simulink model "ArduPlane_LindiPlane"  (R2023b)
settings: Solver=FixedStepDiscrete  StartTime=0.0  StopTime=1000  FixedStep=double(lindi_notune.ts)  RelTol=1e-4
libraries: ardupilot_custom_controller_lib x2, simulink x2, lindiPlane_lib x1, axes_transformation_lib x1
settings Model: DataTypeOverride=Single  DataTypeOverrideAppliesTo=Floating-point  TunableVars=lindi  TunableVarsStorageClass=Auto  Creator=Yannic  LastModifiedBy=yannic
settings SolverCC: ZeroCrossControl=DisableAll  AlgebraicLoopSolver=TrustRegion
settings DataIOCC: LimitDataPoints=on  SaveOutput=off  SaveTime=off
settings OptimizationCC: DefaultParameterBehavior=Inlined  UseDivisionForNetSlopeComputation=on  UseFloatMulNetSlope=on  DefaultUnderspecifiedDataType=single  InlineInvariantSignals=on  ReuseModelBlockBuffer=off  PassReuseOutputArgsAs=Individual arguments  ZeroExternalMemoryAtStartup=off  ZeroInternalMemoryAtStartup=off  NoFixptDivByZeroProtection=on  EfficientFloat2IntCast=on  LifeSpan=1  OptimizationLevel=level1  OptimizationCustomize=off  EfficientTunableParamExpr=on
settings DebuggingCC: ReadBeforeWriteMsg=DisableAll  WriteAfterWriteMsg=DisableAll  WriteAfterReadMsg=DisableAll  MultiTaskDSMMsg=none  ParameterTunabilityLossMsg=error  UnconnectedInputMsg=warning  UnconnectedOutputMsg=warning  UnconnectedLineMsg=warning  AllowSymbolicDim=off  SFUnexpectedBacktrackingDiag=warning  SFNoUnconditionalDefaultTransitionDiag=warning  SFExecutionAtInitializationDiag=none  ArithmeticOperatorsInVariantConditions=warning
settings HardwareCC: ProdBitPerLong=64  ProdLongLongMode=on  ProdHWDeviceType=Intel->x86-64 (Linux 64)
settings ModelReferenceCC: UpdateModelReferenceTargets=IfOutOfDate  EnableRefExpFcnMdlSchedulingChecks=on  PropagateSignalLabelsOutOfModel=off
settings SFSimCC: SFSimEcho=off  SimUseLocalCustomCode=off  MATLABDynamicMemAlloc=off  CustomCodeUndefinedFunction=UseInterfaceOnly  SimTargetLang=C++
settings RTWCC: Description=Embedded Coder  SystemTargetFile=ert.tlc  GenCodeOnly=on  TemplateMakefile=ert_default_tmf  GenerateReport=on  RTWUseLocalCustomCode=off  CustomSourceCode=//custom_source_file_import_identifier  CustomHeaderCode=//custom_header_file_import_identifier  IncludeHyperlinkInReport=on  LaunchReport=on  TargetLang=C++  GenerateTraceInfo=on  GenerateTraceReport=on  GenerateTraceReportSl=on  GenerateTraceReportSf=on  GenerateTraceReportEml=on
settings CodeAppCC: ForceParamTrailComments=on  IgnoreCustomStorageClasses=off  OperatorAnnotations=on  SimulinkDataObjDesc=on  SFDataObjDesc=on  CustomSymbolStrGlobalVar=rt$N$M  CustomSymbolStrType=$N$M  CustomSymbolStrFcn=$N$M$F  CustomSymbolStrMacro=$N$M  InsertBlockDesc=on
settings ERTTargetCC: TargetLangStandard=C++03 (ISO)  IncludeMdlTerminateFcn=off  CombineSignalStateStructs=on  SuppressErrorStatus=on  SupportAbsoluteTime=off  CodeInterfacePackaging=C++ class  SupportNonFinite=off  SupportComplex=off  SupportVariableSizeSignals=on  ERTHeaderFileRootName=MatlabController$E  ERTSourceFileRootName=MatlabController$E  ERTDataFileRootName=MatlabController_data  InlinedParameterPlacement=NonHierarchical  RootIOFormat=Structure reference  ERTCustomFileTemplate=example_file_process.tlc  ERTFilePackagingFormat=CompactWithDataFile
settings ConfigComp: CovMetricSettings=dw  CovSaveCumulativeToWorkspaceVar=on  CovSaveSingleToWorkspaceVar=on  CovExternalEMLEnable=off

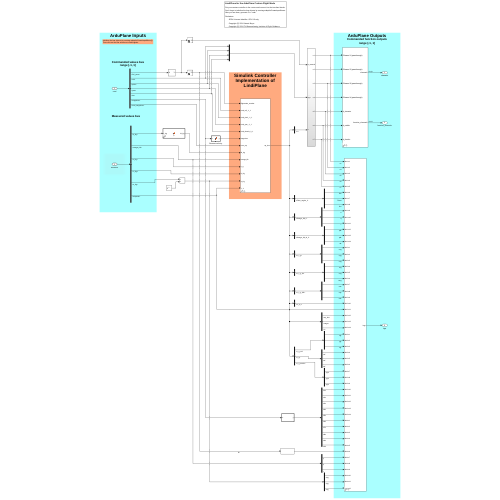
[thumbnail: Simulink's stored preview of the top-level diagram]
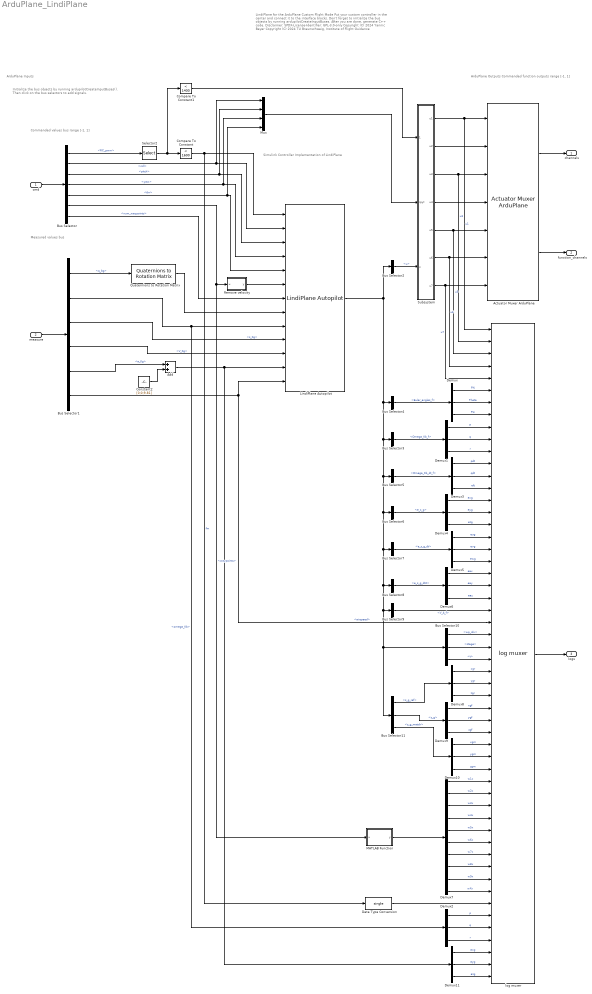
== system ArduPlane_LindiPlane ==
  note: Measured values bus
  note: Initialize the bus objects by running ardupilotCreateInputBuses().
      | Then click on the bus selectors to add signals.
  note: Commanded values bus
      | range [-1, 1]
  note: ArduPlane Inputs
  note: ArduPlane Outputs
      | Commanded function outputs
      | range [-1, 1]
  note: Simulink Controller
      | Implementation of
      | LindiPlane
  note: LindiPlane for the ArduPlane Custom Flight Mode
      |
      | Put your custom controller in the center and connect it to the interface blocks.
      | Don't forget to initialize the bus objects by running ardupilotCreateInputBuses.
      | After you are done, generate C++ code.
      |
      | Disclaimer:
      | SPDX-License-Identifier: GPL-3.0-only
      |
      | Copyright (C) 2024 Yannic Beyer
      | Copyright (C) 2024 TU Braunschweig, Institute of Flight Guidance
  cmd : Inport  OutDataTypeStr=Bus: cmdBus
  measure : Inport  Port=2  OutDataTypeStr=Bus: measureBus
  Actuator Muxer ArduPlane : ardupilot_custom_controller_lib/Actuator Muxer ArduPlane  num_channels=7  CHFCN1=passthrough  CHFCN2=passthrough  CHFCN3=passthrough  CHFCN4=passthrough  CHFCN5=k_elevator  CHFCN6=k_rudder  CHFCN7=k_throttle  CHFCN8=passthrough  CHFCN9=k_elevator  CHFCN10=k_rudder  CHFCN11=k_throttle  CHFCN12=k_none  CHFCN13=k_none  CHFCN14=k_none  CHFCN15=k_none  CHFCN16=k_none
      settings: SourceProductName=LADAC
  Add : Sum
  Bus Selector : BusSelector  OutputSignals=RC_pwm,roll,pitch,yaw,thr,waypoints,num_waypoints
  Bus Selector1 : BusSelector  OutputSignals=q_bg,omega_Kb,s_Kg,V_Kg,a_Kg,airspeed
  Bus Selector10 : BusSelector  OutputSignals=wpnav.wp_idx,wpnav.stage,wpnav.t
  Bus Selector11 : BusSelector  OutputSignals=pos_control.reference.s_g_ref,pos_control.measure.s_g,wpnav.s_g_match
  Bus Selector2 : BusSelector  OutputSignals=inner_loop_indi.u
  Bus Selector3 : BusSelector  OutputSignals=measurements.Omega_Kb_f
  Bus Selector4 : BusSelector  OutputSignals=measurements.Euler_angles_f
  Bus Selector5 : BusSelector  OutputSignals=measurements.Omega_Kb_dt_f
  Bus Selector6 : BusSelector  OutputSignals=pos_control.error.e_s_g
  Bus Selector7 : BusSelector  OutputSignals=pos_control.error.e_s_g_dt
  Bus Selector8 : BusSelector  OutputSignals=pos_control.error.e_s_g_dt2
  Bus Selector9 : BusSelector  OutputSignals=measurements.V_A_f
  Compare To Constant : simulink/Logic and Bit Operations/Compare To Constant  relop=<  const=1600  OutDataTypeStr=uint8
  Compare To Constant1 : simulink/Logic and Bit Operations/Compare To Constant  relop=<  const=1400  OutDataTypeStr=boolean
  Constant2 : Constant  Value=[0;0;9.81]  OutDataTypeStr=Inherit: Inherit via back propagation
  Data Type Conversion : DataTypeConversion  OutDataTypeStr=single  SaturateOnIntegerOverflow=off  RndMeth=Floor
  Demux{,1..6,8..11} (11 alike) : Demux  Outputs=3
  Demux7 : Demux  Outputs=10
  LindiPlane Autopilot : lindiPlane_lib/LindiPlane Autopilot  ap=lindi  ap_notune=lindi_notune  is_enable_checked=off  states_when_enabling=reset  is_cmd_wrbm_n=off
  MATLAB Function : MATLAB Function  TreatAsAtomicUnit=on
  Mux : Mux
  Quaternions to Rotation Matrix : axes_transformation_lib/Quaternions to Rotation Matrix  SystemSampleTime=-1  VariantActivationTime=update diagram  AllowFlexibleInterface=on  Latency=0  AutoFrameSizeCalculation=off
      settings: SourceProductName=LADAC
  Remove velocity : MATLAB Function  TreatAsAtomicUnit=on
  Selector2 : Selector  InputPortWidth=16  IndexOptions=Index vector (dialog)  Indices=8  OutputSizes=1
  Subsystem : Subsystem
  log muxer : ardupilot_custom_controller_lib/log muxer  batch_name_1='ML1'  num_signals_1=14  batch_name_2='ML2'  num_signals_2=14  batch_name_3='ML3'  num_signals_3=14  batch_name_4='ML4'  num_signals_4=12  batch_name_5='ML5'  num_signals_5=0
      settings: SourceProductName=LADAC
  channels : Outport  VectorParamsAs1DForOutWhenUnconnected=off
  function_channels : Outport  Port=2  VectorParamsAs1DForOutWhenUnconnected=off
  logs : Outport  Port=3  VectorParamsAs1DForOutWhenUnconnected=off
  wires:
  cmd/1 -> Bus Selector/1
  measure/1 -> Bus Selector1/1
  Bus Selector1/2 -> LindiPlane Autopilot/9, Demux2/1  "<omega_Kb>"
  Bus Selector/2 -> LindiPlane Autopilot/2, Mux/1  "<roll>"
  Bus Selector/3 -> LindiPlane Autopilot/3, Mux/2  "<pitch>"
  Bus Selector/4 -> LindiPlane Autopilot/4, Mux/3  "<yaw>"
  Bus Selector/5 -> LindiPlane Autopilot/5, Mux/4  "<thr>"
  Bus Selector1/4 -> LindiPlane Autopilot/11  "<V_Kg>"
  log muxer/1 -> logs/1
  Demux/1 -> log muxer/6  "Phi"
  Demux/2 -> log muxer/7  "Theta"
  Demux/3 -> log muxer/8  "Psi"
  Demux1/1 -> log muxer/9  "p"
  Demux1/2 -> log muxer/10  "q"
  Demux1/3 -> log muxer/11  "r"
  Demux3/1 -> log muxer/12  "pdt"
  Demux3/2 -> log muxer/13  "qdt"
  Demux3/3 -> log muxer/14  "rdt"
  Actuator Muxer ArduPlane/1 -> channels/1
  Actuator Muxer ArduPlane/2 -> function_channels/1
  Bus Selector1/1 -> Quaternions to Rotation Matrix/1  "<q_bg>"
  Quaternions to Rotation Matrix/1 -> LindiPlane Autopilot/8
  Bus Selector1/3 -> LindiPlane Autopilot/10  "<s_Kg>"
  Bus Selector1/5 -> Add/1  "<a_Kg>"
  Bus Selector1/6 -> LindiPlane Autopilot/13, log muxer/25  "<airspeed>"
  Bus Selector/6 -> MATLAB Function/1(u), Remove velocity/1(u)  "<waypoints>"
  LindiPlane Autopilot/1 -> Bus Selector11/1, Bus Selector10/1, Bus Selector9/1, Bus Selector8/1, Bus Selector7/1, Bus Selector6/1, Bus Selector5/1, Bus Selector3/1, Bus Selector4/1, Bus Selector2/1
  Bus Selector4/1 -> Demux/1  "<Euler_angles_f>"
  Bus Selector3/1 -> Demux1/1  "<Omega_Kb_f>"
  Bus Selector5/1 -> Demux3/1  "<Omega_Kb_dt_f>"
  Demux4/1 -> log muxer/15  "exg"
  Demux4/2 -> log muxer/16  "eyg"
  Demux4/3 -> log muxer/17  "ezg"
  Bus Selector6/1 -> Demux4/1  "<e_s_g>"
  Demux5/1 -> log muxer/18  "eug"
  Demux5/2 -> log muxer/19  "evg"
  Demux5/3 -> log muxer/20  "ewg"
  Bus Selector7/1 -> Demux5/1  "<e_s_g_dt>"
  Demux6/1 -> log muxer/21  "eax"
  Demux6/2 -> log muxer/22  "eay"
  Demux6/3 -> log muxer/23  "eaz"
  Bus Selector8/1 -> Demux6/1  "<e_s_g_dt2>"
  Bus Selector9/1 -> log muxer/24  "<V_A_f>"
  Bus Selector/1 -> Selector2/1  "<RC_pwm>"
  Compare To Constant/1 -> LindiPlane Autopilot/1, Data Type Conversion/1  "fm"
  Remove velocity/1(y) -> LindiPlane Autopilot/6
  Selector2/1 -> Compare To Constant1/1, Compare To Constant/1
  Bus Selector2/1 -> Subsystem/3(u)  "<u>"
  Subsystem/7(u7) -> log muxer/5, Actuator Muxer ArduPlane/7  "u7"
  Subsystem/4(u4) -> Actuator Muxer ArduPlane/4
  Subsystem/3(u3) -> log muxer/2, Actuator Muxer ArduPlane/3  "u3"
  Subsystem/2(u2) -> Actuator Muxer ArduPlane/2
  Subsystem/1(u1) -> Actuator Muxer ArduPlane/1, log muxer/1  "u1"
  Subsystem/5(u5) -> log muxer/3, Actuator Muxer ArduPlane/5  "u5"
  Subsystem/6(u6) -> log muxer/4, Actuator Muxer ArduPlane/6  "u6"
  Mux/1 -> Subsystem/2(rpyt)
  Compare To Constant1/1 -> Subsystem/1(is_manual)
  MATLAB Function/1(y) -> Demux7/1
  Constant2/1 -> Add/2
  Add/1 -> Demux11/1, LindiPlane Autopilot/12
  Demux2/3 -> log muxer/51  "r"
  Demux2/2 -> log muxer/50  "q"
  Demux2/1 -> log muxer/49  "p"
  Demux7/10 -> log muxer/47  "wXx"
  Demux7/9 -> log muxer/46  "w9x"
  Demux7/8 -> log muxer/45  "w8x"
  Demux7/7 -> log muxer/44  "w7x"
  Demux7/6 -> log muxer/43  "w6x"
  Demux7/5 -> log muxer/42  "w5x"
  Demux7/4 -> log muxer/41  "w4x"
  Demux7/3 -> log muxer/40  "w3x"
  Demux7/2 -> log muxer/39  "w2x"
  Demux7/1 -> log muxer/38  "w1x"
  Data Type Conversion/1 -> log muxer/48
  Bus Selector10/1 -> log muxer/26  "<wp_idx>"
  Bus Selector10/2 -> log muxer/27  "<stage>"
  Bus Selector10/3 -> log muxer/28  "<t>"
  Bus Selector11/1 -> Demux8/1  "<s_g_ref>"
  Demux8/1 -> log muxer/29  "xgr"
  Demux8/2 -> log muxer/30  "ygr"
  Demux8/3 -> log muxer/31  "zgr"
  Demux9/1 -> log muxer/32  "xgf"
  Demux9/2 -> log muxer/33  "ygf"
  Demux9/3 -> log muxer/34  "zgf"
  Bus Selector11/2 -> Demux9/1  "<s_g>"
  Demux10/1 -> log muxer/35  "xgm"
  Demux10/2 -> log muxer/36  "ygm"
  Demux10/3 -> log muxer/37  "zgm"
  Bus Selector11/3 -> Demux10/1  "<s_g_match>"
  Bus Selector/7 -> LindiPlane Autopilot/7  "<num_waypoints>"
  Demux11/3 -> log muxer/54  "azg"
  Demux11/2 -> log muxer/53  "ayg"
  Demux11/1 -> log muxer/52  "axg"

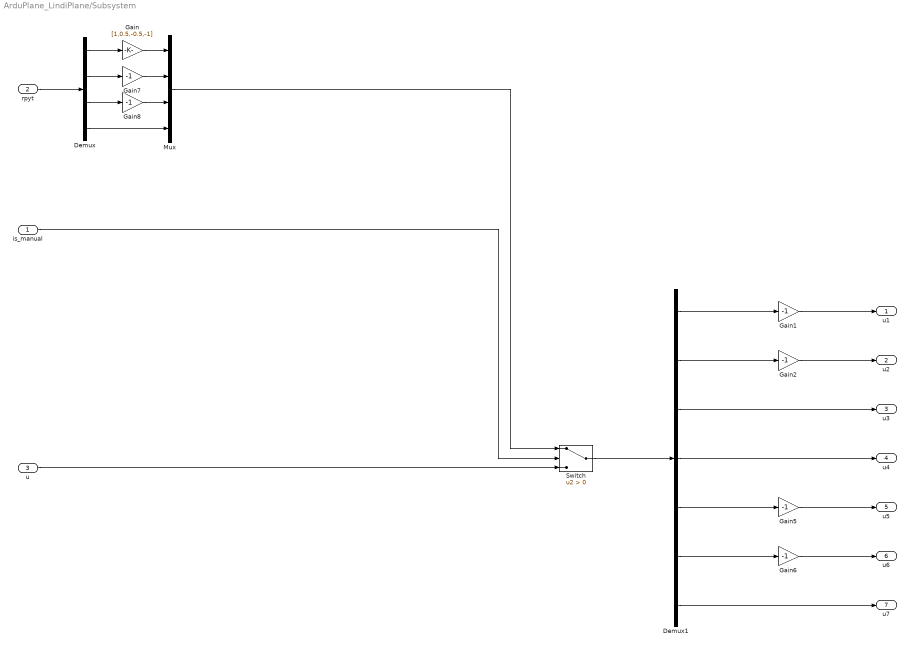
== system ArduPlane_LindiPlane/Subsystem ==
  is_manual : Inport
  rpyt : Inport  Port=2
  u : Inport  Port=3
  Demux : Demux
  Demux1 : Demux  Outputs=7
  Gain : Gain  Gain=[1,0.5,-0.5,-1]
  Gain{1..2,5..8} (6 alike) : Gain  Gain=-1
  Mux : Mux
  Switch : Switch  Criteria=u2 > Threshold  SaturateOnIntegerOverflow=off  InputSameDT=off
  u1 : Outport  VectorParamsAs1DForOutWhenUnconnected=off
  u2 : Outport  Port=2  VectorParamsAs1DForOutWhenUnconnected=off
  u3 : Outport  Port=3  VectorParamsAs1DForOutWhenUnconnected=off
  u4 : Outport  Port=4  VectorParamsAs1DForOutWhenUnconnected=off
  u5 : Outport  Port=5  VectorParamsAs1DForOutWhenUnconnected=off
  u6 : Outport  Port=6  VectorParamsAs1DForOutWhenUnconnected=off
  u7 : Outport  Port=7  VectorParamsAs1DForOutWhenUnconnected=off
  wires:
  is_manual/1 -> Switch/2
  rpyt/1 -> Demux/1
  Demux/1 -> Gain/1
  Demux/4 -> Mux/4
  Demux/3 -> Gain8/1
  Demux/2 -> Gain7/1
  Gain/1 -> Mux/1
  Mux/1 -> Switch/1
  Demux1/1 -> Gain1/1
  Demux1/2 -> Gain2/1
  Demux1/7 -> u7/1
  Demux1/6 -> Gain6/1
  Demux1/5 -> Gain5/1
  Demux1/4 -> u4/1
  Demux1/3 -> u3/1
  u/1 -> Switch/3
  Gain1/1 -> u1/1
  Gain2/1 -> u2/1
  Switch/1 -> Demux1/1
  Gain5/1 -> u5/1
  Gain6/1 -> u6/1
  Gain7/1 -> Mux/2
  Gain8/1 -> Mux/3

== matlab function ArduPlane_LindiPlane/MATLAB Function ==
  data: u input; y output
function y = fcn(u)

y = u(1,:);

== matlab function ArduPlane_LindiPlane/Remove velocity ==
  data: u input; y output
function y = fcn(u)
y = u(1:3,:);
end
